simulink model "CabinGuard_MATLAB_simulation"  (R2024a)
settings: Solver=ode4  StartTime=0.0  StopTime=45  FixedStep=0.01  RelTol=1e-3
undefined symbols (not defined in the file or in its folder): ca_a_comf, ca_a_lo, ca_absvel, ca_clear, ca_d0, ca_det, ca_edge, ca_ego_id, ca_go_phase, ca_hw, ca_jdn, ca_jup, ca_kfeas, ca_lka_in, ca_lka_out, ca_lw0, ca_min_shift, ca_plant, ca_psi0, ca_pv, ca_sys, ca_t_act, ca_v0, ca_vlat, ca_wn, ca_X0, ca_Y0, driving, matlabshared
libraries: simulink x102, drivingscenarioandsensors x5, autolibshared x2, mpcadaslib x1, slpidlib x1
(part 4 of 4)

== system CabinGuard_MATLAB_simulation/GNC/Perception/C2_4 ==
  x : Inport
  y : Inport  Port=2
  vx : Inport  Port=3
  vy : Inport  Port=4
  v : Inport  Port=5
  kap : Inport  Port=6
  vm : Inport  Port=7
  xf : Inport  Port=8
  ASw : Switch  Criteria=u2 ~= 0  SaturateOnIntegerOverflow=off  InputSameDT=off
  AbsK : Constant  Value=ca_absvel
  AbsVm : Product  Inputs=**
  AbsY : Abs  SaturateOnIntegerOverflow=off
  Areq0 : Product  Inputs=*/
  B12 : Constant  Value=12
  Bsum : Sum
  D0 : Constant  Value=ca_d0
  Dx : Sum  Inputs=+-
  DxS : Saturate  UpperLimit=inf  LowerLimit=0.5
  G3 : Gain  Gain=3
  Half : Gain  Gain=0.5
  HalfA : Gain  Gain=0.5
  InPath : Logic  Inputs=3  AllPortsSameDT=off  OutDataTypeStr=boolean
  InW : simulink/Logic and Bit Operations/Compare To Constant  relop=<  const=ca_hw  OutDataTypeStr=boolean
  KX2 : Product  Inputs=**
  NegB : Gain  Gain=-1
  NegVx : Gain  Gain=-1
  Occ : Logic  Inputs=5  AllPortsSameDT=off  OutDataTypeStr=boolean
  Tm : Product  Inputs=*/
  Vc : Saturate  UpperLimit=inf  LowerLimit=0
  Vc2 : Product  Inputs=**
  VmS : Saturate  UpperLimit=inf  LowerLimit=1
  VxP : Saturate  UpperLimit=inf  LowerLimit=0
  VxRel : Sum  Inputs=+-
  VyT : Product  Inputs=**
  X2 : Product  Inputs=**
  XB : RelationalOperator  Operator=>  OutDataTypeStr=boolean  RndMeth=Simplest  InputSameDT=off
  XL : RelationalOperator  Operator=<  OutDataTypeStr=boolean  RndMeth=Simplest  InputSameDT=off
  XPos : simulink/Logic and Bit Operations/Compare To Constant  relop=>  const=0.5  OutDataTypeStr=boolean
  YP : Sum  Inputs=+-
  YPred : Sum
  YR1 : simulink/Logic and Bit Operations/Compare To Constant  relop=<  const=-0.9  OutDataTypeStr=boolean
  YR2 : simulink/Logic and Bit Operations/Compare To Constant  relop=>  const=-ca_clear+0.2  OutDataTypeStr=boolean
  Zero : Constant  Value=0
  areq : Outport
  occ : Outport  Port=2
  wires:
  AbsK/1 -> AbsVm/2
  xf/1 -> XL/2
  vm/1 -> VmS/1, AbsVm/1
  VxRel/1 -> NegVx/1, VxP/1
  vy/1 -> VyT/1
  vx/1 -> VxRel/1
  D0/1 -> Dx/2
  AbsVm/1 -> VxRel/2
  VmS/1 -> Tm/2
  ASw/1 -> areq/1
  y/1 -> YP/1
  x/1 -> Dx/1, XB/1, XPos/1, Tm/1, X2/2, XL/1, X2/1
  NegVx/1 -> Vc/1
  DxS/1 -> Areq0/2
  Dx/1 -> DxS/1
  Tm/1 -> VyT/2
  v/1 -> InPath/1, Occ/1
  kap/1 -> KX2/1
  X2/1 -> KX2/2
  VxP/1 -> G3/1
  YR2/1 -> Occ/3
  YR1/1 -> Occ/2
  XL/1 -> Occ/4
  Vc/1 -> Vc2/2, Vc2/1
  VyT/1 -> YPred/2
  NegB/1 -> XB/2
  KX2/1 -> Half/1
  G3/1 -> Bsum/1
  Areq0/1 -> HalfA/1
  B12/1 -> Bsum/2
  Vc2/1 -> Areq0/1
  Half/1 -> YP/2
  AbsY/1 -> InW/1
  Bsum/1 -> NegB/1
  YP/1 -> YPred/1, YR2/1, YR1/1
  YPred/1 -> AbsY/1
  XB/1 -> Occ/5
  Zero/1 -> ASw/3
  XPos/1 -> InPath/2
  Occ/1 -> occ/1
  HalfA/1 -> ASw/1
  InW/1 -> InPath/3
  InPath/1 -> ASw/2

== system CabinGuard_MATLAB_simulation/GNC/Perception/C2_5 ==
  x : Inport
  y : Inport  Port=2
  vx : Inport  Port=3
  vy : Inport  Port=4
  v : Inport  Port=5
  kap : Inport  Port=6
  vm : Inport  Port=7
  xf : Inport  Port=8
  ASw : Switch  Criteria=u2 ~= 0  SaturateOnIntegerOverflow=off  InputSameDT=off
  AbsK : Constant  Value=ca_absvel
  AbsVm : Product  Inputs=**
  AbsY : Abs  SaturateOnIntegerOverflow=off
  Areq0 : Product  Inputs=*/
  B12 : Constant  Value=12
  Bsum : Sum
  D0 : Constant  Value=ca_d0
  Dx : Sum  Inputs=+-
  DxS : Saturate  UpperLimit=inf  LowerLimit=0.5
  G3 : Gain  Gain=3
  Half : Gain  Gain=0.5
  HalfA : Gain  Gain=0.5
  InPath : Logic  Inputs=3  AllPortsSameDT=off  OutDataTypeStr=boolean
  InW : simulink/Logic and Bit Operations/Compare To Constant  relop=<  const=ca_hw  OutDataTypeStr=boolean
  KX2 : Product  Inputs=**
  NegB : Gain  Gain=-1
  NegVx : Gain  Gain=-1
  Occ : Logic  Inputs=5  AllPortsSameDT=off  OutDataTypeStr=boolean
  Tm : Product  Inputs=*/
  Vc : Saturate  UpperLimit=inf  LowerLimit=0
  Vc2 : Product  Inputs=**
  VmS : Saturate  UpperLimit=inf  LowerLimit=1
  VxP : Saturate  UpperLimit=inf  LowerLimit=0
  VxRel : Sum  Inputs=+-
  VyT : Product  Inputs=**
  X2 : Product  Inputs=**
  XB : RelationalOperator  Operator=>  OutDataTypeStr=boolean  RndMeth=Simplest  InputSameDT=off
  XL : RelationalOperator  Operator=<  OutDataTypeStr=boolean  RndMeth=Simplest  InputSameDT=off
  XPos : simulink/Logic and Bit Operations/Compare To Constant  relop=>  const=0.5  OutDataTypeStr=boolean
  YP : Sum  Inputs=+-
  YPred : Sum
  YR1 : simulink/Logic and Bit Operations/Compare To Constant  relop=<  const=-0.9  OutDataTypeStr=boolean
  YR2 : simulink/Logic and Bit Operations/Compare To Constant  relop=>  const=-ca_clear+0.2  OutDataTypeStr=boolean
  Zero : Constant  Value=0
  areq : Outport
  occ : Outport  Port=2
  wires:
  x/1 -> Dx/1, XB/1, XL/1, XPos/1, X2/2, Tm/1, X2/1
  VxRel/1 -> VxP/1, NegVx/1
  X2/1 -> KX2/2
  AbsK/1 -> AbsVm/2
  y/1 -> YP/1
  vx/1 -> VxRel/1
  kap/1 -> KX2/1
  vm/1 -> AbsVm/1, VmS/1
  AbsY/1 -> InW/1
  AbsVm/1 -> VxRel/2
  VmS/1 -> Tm/2
  Bsum/1 -> NegB/1
  D0/1 -> Dx/2
  xf/1 -> XL/2
  NegVx/1 -> Vc/1
  Dx/1 -> DxS/1
  vy/1 -> VyT/1
  Vc/1 -> Vc2/2, Vc2/1
  Tm/1 -> VyT/2
  VxP/1 -> G3/1
  XL/1 -> Occ/4
  VyT/1 -> YPred/2
  KX2/1 -> Half/1
  G3/1 -> Bsum/1
  B12/1 -> Bsum/2
  Vc2/1 -> Areq0/1
  DxS/1 -> Areq0/2
  InW/1 -> InPath/3
  HalfA/1 -> ASw/1
  Half/1 -> YP/2
  Areq0/1 -> HalfA/1
  YP/1 -> YPred/1, YR2/1, YR1/1
  NegB/1 -> XB/2
  v/1 -> InPath/1, Occ/1
  YR1/1 -> Occ/2
  YPred/1 -> AbsY/1
  YR2/1 -> Occ/3
  XB/1 -> Occ/5
  Occ/1 -> occ/1
  XPos/1 -> InPath/2
  InPath/1 -> ASw/2
  Zero/1 -> ASw/3
  ASw/1 -> areq/1

== system CabinGuard_MATLAB_simulation/GNC/Perception/C2_6 ==
  x : Inport
  y : Inport  Port=2
  vx : Inport  Port=3
  vy : Inport  Port=4
  v : Inport  Port=5
  kap : Inport  Port=6
  vm : Inport  Port=7
  xf : Inport  Port=8
  ASw : Switch  Criteria=u2 ~= 0  SaturateOnIntegerOverflow=off  InputSameDT=off
  AbsK : Constant  Value=ca_absvel
  AbsVm : Product  Inputs=**
  AbsY : Abs  SaturateOnIntegerOverflow=off
  Areq0 : Product  Inputs=*/
  B12 : Constant  Value=12
  Bsum : Sum
  D0 : Constant  Value=ca_d0
  Dx : Sum  Inputs=+-
  DxS : Saturate  UpperLimit=inf  LowerLimit=0.5
  G3 : Gain  Gain=3
  Half : Gain  Gain=0.5
  HalfA : Gain  Gain=0.5
  InPath : Logic  Inputs=3  AllPortsSameDT=off  OutDataTypeStr=boolean
  InW : simulink/Logic and Bit Operations/Compare To Constant  relop=<  const=ca_hw  OutDataTypeStr=boolean
  KX2 : Product  Inputs=**
  NegB : Gain  Gain=-1
  NegVx : Gain  Gain=-1
  Occ : Logic  Inputs=5  AllPortsSameDT=off  OutDataTypeStr=boolean
  Tm : Product  Inputs=*/
  Vc : Saturate  UpperLimit=inf  LowerLimit=0
  Vc2 : Product  Inputs=**
  VmS : Saturate  UpperLimit=inf  LowerLimit=1
  VxP : Saturate  UpperLimit=inf  LowerLimit=0
  VxRel : Sum  Inputs=+-
  VyT : Product  Inputs=**
  X2 : Product  Inputs=**
  XB : RelationalOperator  Operator=>  OutDataTypeStr=boolean  RndMeth=Simplest  InputSameDT=off
  XL : RelationalOperator  Operator=<  OutDataTypeStr=boolean  RndMeth=Simplest  InputSameDT=off
  XPos : simulink/Logic and Bit Operations/Compare To Constant  relop=>  const=0.5  OutDataTypeStr=boolean
  YP : Sum  Inputs=+-
  YPred : Sum
  YR1 : simulink/Logic and Bit Operations/Compare To Constant  relop=<  const=-0.9  OutDataTypeStr=boolean
  YR2 : simulink/Logic and Bit Operations/Compare To Constant  relop=>  const=-ca_clear+0.2  OutDataTypeStr=boolean
  Zero : Constant  Value=0
  areq : Outport
  occ : Outport  Port=2
  wires:
  AbsK/1 -> AbsVm/2
  kap/1 -> KX2/1
  vm/1 -> AbsVm/1, VmS/1
  x/1 -> Dx/1, XB/1, XL/1, Tm/1, XPos/1, X2/1, X2/2
  y/1 -> YP/1
  vx/1 -> VxRel/1
  DxS/1 -> Areq0/2
  AbsVm/1 -> VxRel/2
  VmS/1 -> Tm/2
  Vc/1 -> Vc2/2, Vc2/1
  D0/1 -> Dx/2
  VxRel/1 -> VxP/1, NegVx/1
  NegB/1 -> XB/2
  xf/1 -> XL/2
  InPath/1 -> ASw/2
  NegVx/1 -> Vc/1
  Dx/1 -> DxS/1
  v/1 -> InPath/1, Occ/1
  vy/1 -> VyT/1
  VyT/1 -> YPred/2
  Tm/1 -> VyT/2
  X2/1 -> KX2/2
  VxP/1 -> G3/1
  InW/1 -> InPath/3
  Occ/1 -> occ/1
  XL/1 -> Occ/4
  YP/1 -> YPred/1, YR2/1, YR1/1
  KX2/1 -> Half/1
  Half/1 -> YP/2
  G3/1 -> Bsum/1
  B12/1 -> Bsum/2
  ASw/1 -> areq/1
  Vc2/1 -> Areq0/1
  Bsum/1 -> NegB/1
  Areq0/1 -> HalfA/1
  YPred/1 -> AbsY/1
  YR1/1 -> Occ/2
  Zero/1 -> ASw/3
  YR2/1 -> Occ/3
  XB/1 -> Occ/5
  XPos/1 -> InPath/2
  AbsY/1 -> InW/1
  HalfA/1 -> ASw/1

== system CabinGuard_MATLAB_simulation/GNC/Perception/C3_1 ==
  x : Inport
  y : Inport  Port=2
  vx : Inport  Port=3
  vy : Inport  Port=4
  v : Inport  Port=5
  kap : Inport  Port=6
  vm : Inport  Port=7
  xf : Inport  Port=8
  ASw : Switch  Criteria=u2 ~= 0  SaturateOnIntegerOverflow=off  InputSameDT=off
  AbsK : Constant  Value=ca_absvel
  AbsVm : Product  Inputs=**
  AbsY : Abs  SaturateOnIntegerOverflow=off
  Areq0 : Product  Inputs=*/
  B12 : Constant  Value=12
  Bsum : Sum
  D0 : Constant  Value=ca_d0
  Dx : Sum  Inputs=+-
  DxS : Saturate  UpperLimit=inf  LowerLimit=0.5
  G3 : Gain  Gain=3
  Half : Gain  Gain=0.5
  HalfA : Gain  Gain=0.5
  InPath : Logic  Inputs=3  AllPortsSameDT=off  OutDataTypeStr=boolean
  InW : simulink/Logic and Bit Operations/Compare To Constant  relop=<  const=ca_hw  OutDataTypeStr=boolean
  KX2 : Product  Inputs=**
  NegB : Gain  Gain=-1
  NegVx : Gain  Gain=-1
  Occ : Logic  Inputs=5  AllPortsSameDT=off  OutDataTypeStr=boolean
  Tm : Product  Inputs=*/
  Vc : Saturate  UpperLimit=inf  LowerLimit=0
  Vc2 : Product  Inputs=**
  VmS : Saturate  UpperLimit=inf  LowerLimit=1
  VxP : Saturate  UpperLimit=inf  LowerLimit=0
  VxRel : Sum  Inputs=+-
  VyT : Product  Inputs=**
  X2 : Product  Inputs=**
  XB : RelationalOperator  Operator=>  OutDataTypeStr=boolean  RndMeth=Simplest  InputSameDT=off
  XL : RelationalOperator  Operator=<  OutDataTypeStr=boolean  RndMeth=Simplest  InputSameDT=off
  XPos : simulink/Logic and Bit Operations/Compare To Constant  relop=>  const=0.5  OutDataTypeStr=boolean
  YP : Sum  Inputs=+-
  YPred : Sum
  YR1 : simulink/Logic and Bit Operations/Compare To Constant  relop=<  const=-0.9  OutDataTypeStr=boolean
  YR2 : simulink/Logic and Bit Operations/Compare To Constant  relop=>  const=-ca_clear+0.2  OutDataTypeStr=boolean
  Zero : Constant  Value=0
  areq : Outport
  occ : Outport  Port=2
  wires:
  VxRel/1 -> VxP/1, NegVx/1
  x/1 -> Dx/1, XPos/1, Tm/1, XB/1, X2/2, X2/1, XL/1
  InW/1 -> InPath/3
  AbsK/1 -> AbsVm/2
  y/1 -> YP/1
  Vc2/1 -> Areq0/1
  vx/1 -> VxRel/1
  KX2/1 -> Half/1
  vm/1 -> VmS/1, AbsVm/1
  AbsY/1 -> InW/1
  AbsVm/1 -> VxRel/2
  VmS/1 -> Tm/2
  Bsum/1 -> NegB/1
  D0/1 -> Dx/2
  NegB/1 -> XB/2
  xf/1 -> XL/2
  NegVx/1 -> Vc/1
  XB/1 -> Occ/5
  Dx/1 -> DxS/1
  Occ/1 -> occ/1
  vy/1 -> VyT/1
  Vc/1 -> Vc2/2, Vc2/1
  Tm/1 -> VyT/2
  YR1/1 -> Occ/2
  YPred/1 -> AbsY/1
  kap/1 -> KX2/1
  YR2/1 -> Occ/3
  X2/1 -> KX2/2
  Zero/1 -> ASw/3
  VxP/1 -> G3/1
  XL/1 -> Occ/4
  ASw/1 -> areq/1
  InPath/1 -> ASw/2
  VyT/1 -> YPred/2
  G3/1 -> Bsum/1
  B12/1 -> Bsum/2
  DxS/1 -> Areq0/2
  Half/1 -> YP/2
  Areq0/1 -> HalfA/1
  YP/1 -> YPred/1, YR2/1, YR1/1
  v/1 -> InPath/1, Occ/1
  XPos/1 -> InPath/2
  HalfA/1 -> ASw/1

== system CabinGuard_MATLAB_simulation/GNC/Perception/C3_2 ==
  x : Inport
  y : Inport  Port=2
  vx : Inport  Port=3
  vy : Inport  Port=4
  v : Inport  Port=5
  kap : Inport  Port=6
  vm : Inport  Port=7
  xf : Inport  Port=8
  ASw : Switch  Criteria=u2 ~= 0  SaturateOnIntegerOverflow=off  InputSameDT=off
  AbsK : Constant  Value=ca_absvel
  AbsVm : Product  Inputs=**
  AbsY : Abs  SaturateOnIntegerOverflow=off
  Areq0 : Product  Inputs=*/
  B12 : Constant  Value=12
  Bsum : Sum
  D0 : Constant  Value=ca_d0
  Dx : Sum  Inputs=+-
  DxS : Saturate  UpperLimit=inf  LowerLimit=0.5
  G3 : Gain  Gain=3
  Half : Gain  Gain=0.5
  HalfA : Gain  Gain=0.5
  InPath : Logic  Inputs=3  AllPortsSameDT=off  OutDataTypeStr=boolean
  InW : simulink/Logic and Bit Operations/Compare To Constant  relop=<  const=ca_hw  OutDataTypeStr=boolean
  KX2 : Product  Inputs=**
  NegB : Gain  Gain=-1
  NegVx : Gain  Gain=-1
  Occ : Logic  Inputs=5  AllPortsSameDT=off  OutDataTypeStr=boolean
  Tm : Product  Inputs=*/
  Vc : Saturate  UpperLimit=inf  LowerLimit=0
  Vc2 : Product  Inputs=**
  VmS : Saturate  UpperLimit=inf  LowerLimit=1
  VxP : Saturate  UpperLimit=inf  LowerLimit=0
  VxRel : Sum  Inputs=+-
  VyT : Product  Inputs=**
  X2 : Product  Inputs=**
  XB : RelationalOperator  Operator=>  OutDataTypeStr=boolean  RndMeth=Simplest  InputSameDT=off
  XL : RelationalOperator  Operator=<  OutDataTypeStr=boolean  RndMeth=Simplest  InputSameDT=off
  XPos : simulink/Logic and Bit Operations/Compare To Constant  relop=>  const=0.5  OutDataTypeStr=boolean
  YP : Sum  Inputs=+-
  YPred : Sum
  YR1 : simulink/Logic and Bit Operations/Compare To Constant  relop=<  const=-0.9  OutDataTypeStr=boolean
  YR2 : simulink/Logic and Bit Operations/Compare To Constant  relop=>  const=-ca_clear+0.2  OutDataTypeStr=boolean
  Zero : Constant  Value=0
  areq : Outport
  occ : Outport  Port=2
  wires:
  y/1 -> YP/1
  Tm/1 -> VyT/2
  vx/1 -> VxRel/1
  AbsK/1 -> AbsVm/2
  vm/1 -> AbsVm/1, VmS/1
  HalfA/1 -> ASw/1
  x/1 -> Dx/1, XPos/1, XL/1, X2/2, X2/1, Tm/1, XB/1
  AbsVm/1 -> VxRel/2
  VmS/1 -> Tm/2
  VxP/1 -> G3/1
  X2/1 -> KX2/2
  VxRel/1 -> NegVx/1, VxP/1
  Bsum/1 -> NegB/1
  D0/1 -> Dx/2
  xf/1 -> XL/2
  Occ/1 -> occ/1
  B12/1 -> Bsum/2
  NegVx/1 -> Vc/1
  YP/1 -> YPred/1, YR1/1, YR2/1
  Dx/1 -> DxS/1
  vy/1 -> VyT/1
  kap/1 -> KX2/1
  XB/1 -> Occ/5
  Half/1 -> YP/2
  G3/1 -> Bsum/1
  XL/1 -> Occ/4
  Vc2/1 -> Areq0/1
  Vc/1 -> Vc2/2, Vc2/1
  YR2/1 -> Occ/3
  VyT/1 -> YPred/2
  KX2/1 -> Half/1
  DxS/1 -> Areq0/2
  Areq0/1 -> HalfA/1
  NegB/1 -> XB/2
  v/1 -> InPath/1, Occ/1
  YPred/1 -> AbsY/1
  AbsY/1 -> InW/1
  YR1/1 -> Occ/2
  XPos/1 -> InPath/2
  InW/1 -> InPath/3
  InPath/1 -> ASw/2
  ASw/1 -> areq/1
  Zero/1 -> ASw/3

== system CabinGuard_MATLAB_simulation/GNC/Perception/C3_3 ==
  x : Inport
  y : Inport  Port=2
  vx : Inport  Port=3
  vy : Inport  Port=4
  v : Inport  Port=5
  kap : Inport  Port=6
  vm : Inport  Port=7
  xf : Inport  Port=8
  ASw : Switch  Criteria=u2 ~= 0  SaturateOnIntegerOverflow=off  InputSameDT=off
  AbsK : Constant  Value=ca_absvel
  AbsVm : Product  Inputs=**
  AbsY : Abs  SaturateOnIntegerOverflow=off
  Areq0 : Product  Inputs=*/
  B12 : Constant  Value=12
  Bsum : Sum
  D0 : Constant  Value=ca_d0
  Dx : Sum  Inputs=+-
  DxS : Saturate  UpperLimit=inf  LowerLimit=0.5
  G3 : Gain  Gain=3
  Half : Gain  Gain=0.5
  HalfA : Gain  Gain=0.5
  InPath : Logic  Inputs=3  AllPortsSameDT=off  OutDataTypeStr=boolean
  InW : simulink/Logic and Bit Operations/Compare To Constant  relop=<  const=ca_hw  OutDataTypeStr=boolean
  KX2 : Product  Inputs=**
  NegB : Gain  Gain=-1
  NegVx : Gain  Gain=-1
  Occ : Logic  Inputs=5  AllPortsSameDT=off  OutDataTypeStr=boolean
  Tm : Product  Inputs=*/
  Vc : Saturate  UpperLimit=inf  LowerLimit=0
  Vc2 : Product  Inputs=**
  VmS : Saturate  UpperLimit=inf  LowerLimit=1
  VxP : Saturate  UpperLimit=inf  LowerLimit=0
  VxRel : Sum  Inputs=+-
  VyT : Product  Inputs=**
  X2 : Product  Inputs=**
  XB : RelationalOperator  Operator=>  OutDataTypeStr=boolean  RndMeth=Simplest  InputSameDT=off
  XL : RelationalOperator  Operator=<  OutDataTypeStr=boolean  RndMeth=Simplest  InputSameDT=off
  XPos : simulink/Logic and Bit Operations/Compare To Constant  relop=>  const=0.5  OutDataTypeStr=boolean
  YP : Sum  Inputs=+-
  YPred : Sum
  YR1 : simulink/Logic and Bit Operations/Compare To Constant  relop=<  const=-0.9  OutDataTypeStr=boolean
  YR2 : simulink/Logic and Bit Operations/Compare To Constant  relop=>  const=-ca_clear+0.2  OutDataTypeStr=boolean
  Zero : Constant  Value=0
  areq : Outport
  occ : Outport  Port=2
  wires:
  v/1 -> InPath/1, Occ/1
  vm/1 -> AbsVm/1, VmS/1
  AbsK/1 -> AbsVm/2
  vx/1 -> VxRel/1
  x/1 -> Dx/1, XPos/1, XL/1, Tm/1, XB/1, X2/2, X2/1
  AbsVm/1 -> VxRel/2
  VmS/1 -> Tm/2
  Dx/1 -> DxS/1
  D0/1 -> Dx/2
  XB/1 -> Occ/5
  VyT/1 -> YPred/2
  X2/1 -> KX2/2
  VxRel/1 -> VxP/1, NegVx/1
  kap/1 -> KX2/1
  xf/1 -> XL/2
  Occ/1 -> occ/1
  YR1/1 -> Occ/2
  NegVx/1 -> Vc/1
  y/1 -> YP/1
  vy/1 -> VyT/1
  Tm/1 -> VyT/2
  VxP/1 -> G3/1
  XL/1 -> Occ/4
  Vc2/1 -> Areq0/1
  Vc/1 -> Vc2/2, Vc2/1
  InPath/1 -> ASw/2
  InW/1 -> InPath/3
  HalfA/1 -> ASw/1
  KX2/1 -> Half/1
  G3/1 -> Bsum/1
  B12/1 -> Bsum/2
  DxS/1 -> Areq0/2
  Half/1 -> YP/2
  Bsum/1 -> NegB/1
  AbsY/1 -> InW/1
  Areq0/1 -> HalfA/1
  XPos/1 -> InPath/2
  YPred/1 -> AbsY/1
  NegB/1 -> XB/2
  YP/1 -> YR2/1, YR1/1, YPred/1
  YR2/1 -> Occ/3
  Zero/1 -> ASw/3
  ASw/1 -> areq/1

== system CabinGuard_MATLAB_simulation/GNC/Perception/C3_4 ==
  x : Inport
  y : Inport  Port=2
  vx : Inport  Port=3
  vy : Inport  Port=4
  v : Inport  Port=5
  kap : Inport  Port=6
  vm : Inport  Port=7
  xf : Inport  Port=8
  ASw : Switch  Criteria=u2 ~= 0  SaturateOnIntegerOverflow=off  InputSameDT=off
  AbsK : Constant  Value=ca_absvel
  AbsVm : Product  Inputs=**
  AbsY : Abs  SaturateOnIntegerOverflow=off
  Areq0 : Product  Inputs=*/
  B12 : Constant  Value=12
  Bsum : Sum
  D0 : Constant  Value=ca_d0
  Dx : Sum  Inputs=+-
  DxS : Saturate  UpperLimit=inf  LowerLimit=0.5
  G3 : Gain  Gain=3
  Half : Gain  Gain=0.5
  HalfA : Gain  Gain=0.5
  InPath : Logic  Inputs=3  AllPortsSameDT=off  OutDataTypeStr=boolean
  InW : simulink/Logic and Bit Operations/Compare To Constant  relop=<  const=ca_hw  OutDataTypeStr=boolean
  KX2 : Product  Inputs=**
  NegB : Gain  Gain=-1
  NegVx : Gain  Gain=-1
  Occ : Logic  Inputs=5  AllPortsSameDT=off  OutDataTypeStr=boolean
  Tm : Product  Inputs=*/
  Vc : Saturate  UpperLimit=inf  LowerLimit=0
  Vc2 : Product  Inputs=**
  VmS : Saturate  UpperLimit=inf  LowerLimit=1
  VxP : Saturate  UpperLimit=inf  LowerLimit=0
  VxRel : Sum  Inputs=+-
  VyT : Product  Inputs=**
  X2 : Product  Inputs=**
  XB : RelationalOperator  Operator=>  OutDataTypeStr=boolean  RndMeth=Simplest  InputSameDT=off
  XL : RelationalOperator  Operator=<  OutDataTypeStr=boolean  RndMeth=Simplest  InputSameDT=off
  XPos : simulink/Logic and Bit Operations/Compare To Constant  relop=>  const=0.5  OutDataTypeStr=boolean
  YP : Sum  Inputs=+-
  YPred : Sum
  YR1 : simulink/Logic and Bit Operations/Compare To Constant  relop=<  const=-0.9  OutDataTypeStr=boolean
  YR2 : simulink/Logic and Bit Operations/Compare To Constant  relop=>  const=-ca_clear+0.2  OutDataTypeStr=boolean
  Zero : Constant  Value=0
  areq : Outport
  occ : Outport  Port=2
  wires:
  AbsK/1 -> AbsVm/2
  AbsVm/1 -> VxRel/2
  v/1 -> InPath/1, Occ/1
  vm/1 -> AbsVm/1, VmS/1
  vx/1 -> VxRel/1
  x/1 -> XB/1, XPos/1, XL/1, Tm/1, X2/1, X2/2, Dx/1
  VyT/1 -> YPred/2
  VxP/1 -> G3/1
  X2/1 -> KX2/2
  VxRel/1 -> NegVx/1, VxP/1
  VmS/1 -> Tm/2
  Areq0/1 -> HalfA/1
  Dx/1 -> DxS/1
  D0/1 -> Dx/2
  y/1 -> YP/1
  kap/1 -> KX2/1
  vy/1 -> VyT/1
  xf/1 -> XL/2
  Occ/1 -> occ/1
  NegVx/1 -> Vc/1
  Tm/1 -> VyT/2
  XL/1 -> Occ/4
  DxS/1 -> Areq0/2
  Vc2/1 -> Areq0/1
  Vc/1 -> Vc2/2, Vc2/1
  InW/1 -> InPath/3
  KX2/1 -> Half/1
  G3/1 -> Bsum/1
  Bsum/1 -> NegB/1
  B12/1 -> Bsum/2
  Half/1 -> YP/2
  XPos/1 -> InPath/2
  YP/1 -> YPred/1, YR2/1, YR1/1
  NegB/1 -> XB/2
  YPred/1 -> AbsY/1
  YR1/1 -> Occ/2
  YR2/1 -> Occ/3
  XB/1 -> Occ/5
  AbsY/1 -> InW/1
  InPath/1 -> ASw/2
  HalfA/1 -> ASw/1
  Zero/1 -> ASw/3
  ASw/1 -> areq/1

== system CabinGuard_MATLAB_simulation/GNC/Perception/C3_5 ==
  x : Inport
  y : Inport  Port=2
  vx : Inport  Port=3
  vy : Inport  Port=4
  v : Inport  Port=5
  kap : Inport  Port=6
  vm : Inport  Port=7
  xf : Inport  Port=8
  ASw : Switch  Criteria=u2 ~= 0  SaturateOnIntegerOverflow=off  InputSameDT=off
  AbsK : Constant  Value=ca_absvel
  AbsVm : Product  Inputs=**
  AbsY : Abs  SaturateOnIntegerOverflow=off
  Areq0 : Product  Inputs=*/
  B12 : Constant  Value=12
  Bsum : Sum
  D0 : Constant  Value=ca_d0
  Dx : Sum  Inputs=+-
  DxS : Saturate  UpperLimit=inf  LowerLimit=0.5
  G3 : Gain  Gain=3
  Half : Gain  Gain=0.5
  HalfA : Gain  Gain=0.5
  InPath : Logic  Inputs=3  AllPortsSameDT=off  OutDataTypeStr=boolean
  InW : simulink/Logic and Bit Operations/Compare To Constant  relop=<  const=ca_hw  OutDataTypeStr=boolean
  KX2 : Product  Inputs=**
  NegB : Gain  Gain=-1
  NegVx : Gain  Gain=-1
  Occ : Logic  Inputs=5  AllPortsSameDT=off  OutDataTypeStr=boolean
  Tm : Product  Inputs=*/
  Vc : Saturate  UpperLimit=inf  LowerLimit=0
  Vc2 : Product  Inputs=**
  VmS : Saturate  UpperLimit=inf  LowerLimit=1
  VxP : Saturate  UpperLimit=inf  LowerLimit=0
  VxRel : Sum  Inputs=+-
  VyT : Product  Inputs=**
  X2 : Product  Inputs=**
  XB : RelationalOperator  Operator=>  OutDataTypeStr=boolean  RndMeth=Simplest  InputSameDT=off
  XL : RelationalOperator  Operator=<  OutDataTypeStr=boolean  RndMeth=Simplest  InputSameDT=off
  XPos : simulink/Logic and Bit Operations/Compare To Constant  relop=>  const=0.5  OutDataTypeStr=boolean
  YP : Sum  Inputs=+-
  YPred : Sum
  YR1 : simulink/Logic and Bit Operations/Compare To Constant  relop=<  const=-0.9  OutDataTypeStr=boolean
  YR2 : simulink/Logic and Bit Operations/Compare To Constant  relop=>  const=-ca_clear+0.2  OutDataTypeStr=boolean
  Zero : Constant  Value=0
  areq : Outport
  occ : Outport  Port=2
  wires:
  AbsVm/1 -> VxRel/2
  Half/1 -> YP/2
  AbsK/1 -> AbsVm/2
  Areq0/1 -> HalfA/1
  x/1 -> XB/1, XPos/1, Dx/1, Tm/1, X2/2, XL/1, X2/1
  v/1 -> InPath/1, Occ/1
  D0/1 -> Dx/2
  vx/1 -> VxRel/1
  AbsY/1 -> InW/1
  Dx/1 -> DxS/1
  vm/1 -> AbsVm/1, VmS/1
  VmS/1 -> Tm/2
  XL/1 -> Occ/4
  VxRel/1 -> VxP/1, NegVx/1
  xf/1 -> XL/2
  VyT/1 -> YPred/2
  NegVx/1 -> Vc/1
  Bsum/1 -> NegB/1
  vy/1 -> VyT/1
  Tm/1 -> VyT/2
  kap/1 -> KX2/1
  Occ/1 -> occ/1
  X2/1 -> KX2/2
  XB/1 -> Occ/5
  VxP/1 -> G3/1
  HalfA/1 -> ASw/1
  Vc/1 -> Vc2/2, Vc2/1
  KX2/1 -> Half/1
  y/1 -> YP/1
  B12/1 -> Bsum/2
  G3/1 -> Bsum/1
  InPath/1 -> ASw/2
  Vc2/1 -> Areq0/1
  DxS/1 -> Areq0/2
  YP/1 -> YPred/1, YR2/1, YR1/1
  NegB/1 -> XB/2
  YPred/1 -> AbsY/1
  YR1/1 -> Occ/2
  YR2/1 -> Occ/3
  Zero/1 -> ASw/3
  XPos/1 -> InPath/2
  InW/1 -> InPath/3
  ASw/1 -> areq/1

== system CabinGuard_MATLAB_simulation/GNC/Perception/C3_6 ==
  x : Inport
  y : Inport  Port=2
  vx : Inport  Port=3
  vy : Inport  Port=4
  v : Inport  Port=5
  kap : Inport  Port=6
  vm : Inport  Port=7
  xf : Inport  Port=8
  ASw : Switch  Criteria=u2 ~= 0  SaturateOnIntegerOverflow=off  InputSameDT=off
  AbsK : Constant  Value=ca_absvel
  AbsVm : Product  Inputs=**
  AbsY : Abs  SaturateOnIntegerOverflow=off
  Areq0 : Product  Inputs=*/
  B12 : Constant  Value=12
  Bsum : Sum
  D0 : Constant  Value=ca_d0
  Dx : Sum  Inputs=+-
  DxS : Saturate  UpperLimit=inf  LowerLimit=0.5
  G3 : Gain  Gain=3
  Half : Gain  Gain=0.5
  HalfA : Gain  Gain=0.5
  InPath : Logic  Inputs=3  AllPortsSameDT=off  OutDataTypeStr=boolean
  InW : simulink/Logic and Bit Operations/Compare To Constant  relop=<  const=ca_hw  OutDataTypeStr=boolean
  KX2 : Product  Inputs=**
  NegB : Gain  Gain=-1
  NegVx : Gain  Gain=-1
  Occ : Logic  Inputs=5  AllPortsSameDT=off  OutDataTypeStr=boolean
  Tm : Product  Inputs=*/
  Vc : Saturate  UpperLimit=inf  LowerLimit=0
  Vc2 : Product  Inputs=**
  VmS : Saturate  UpperLimit=inf  LowerLimit=1
  VxP : Saturate  UpperLimit=inf  LowerLimit=0
  VxRel : Sum  Inputs=+-
  VyT : Product  Inputs=**
  X2 : Product  Inputs=**
  XB : RelationalOperator  Operator=>  OutDataTypeStr=boolean  RndMeth=Simplest  InputSameDT=off
  XL : RelationalOperator  Operator=<  OutDataTypeStr=boolean  RndMeth=Simplest  InputSameDT=off
  XPos : simulink/Logic and Bit Operations/Compare To Constant  relop=>  const=0.5  OutDataTypeStr=boolean
  YP : Sum  Inputs=+-
  YPred : Sum
  YR1 : simulink/Logic and Bit Operations/Compare To Constant  relop=<  const=-0.9  OutDataTypeStr=boolean
  YR2 : simulink/Logic and Bit Operations/Compare To Constant  relop=>  const=-ca_clear+0.2  OutDataTypeStr=boolean
  Zero : Constant  Value=0
  areq : Outport
  occ : Outport  Port=2
  wires:
  AbsVm/1 -> VxRel/2
  AbsK/1 -> AbsVm/2
  Areq0/1 -> HalfA/1
  x/1 -> XB/1, XL/1, XPos/1, Dx/1, Tm/1, X2/1, X2/2
  vx/1 -> VxRel/1
  AbsY/1 -> InW/1
  vm/1 -> AbsVm/1, VmS/1
  DxS/1 -> Areq0/2
  VmS/1 -> Tm/2
  HalfA/1 -> ASw/1
  Vc/1 -> Vc2/2, Vc2/1
  D0/1 -> Dx/2
  XL/1 -> Occ/4
  VxRel/1 -> NegVx/1, VxP/1
  xf/1 -> XL/2
  NegVx/1 -> Vc/1
  InPath/1 -> ASw/2
  Vc2/1 -> Areq0/1
  Dx/1 -> DxS/1
  vy/1 -> VyT/1
  Half/1 -> YP/2
  Tm/1 -> VyT/2
  kap/1 -> KX2/1
  X2/1 -> KX2/2
  XB/1 -> Occ/5
  VxP/1 -> G3/1
  VyT/1 -> YPred/2
  KX2/1 -> Half/1
  B12/1 -> Bsum/2
  G3/1 -> Bsum/1
  y/1 -> YP/1
  Bsum/1 -> NegB/1
  YP/1 -> YR2/1, YR1/1, YPred/1
  NegB/1 -> XB/2
  v/1 -> InPath/1, Occ/1
  YPred/1 -> AbsY/1
  YR1/1 -> Occ/2
  YR2/1 -> Occ/3
  Zero/1 -> ASw/3
  XPos/1 -> InPath/2
  Occ/1 -> occ/1
  InW/1 -> InPath/3
  ASw/1 -> areq/1

== matlab function CabinGuard_MATLAB_simulation/CabinGuard/Tel ==
  settings: updateMethod=DISCRETE  sampleTime=0.01
  data: t input; delivered output; ecall input; cls input; Pmax input; cell_up input; sms_up input
function delivered  = fcn(t, ecall, cls, Pmax, cell_up, sms_up)
% EMERGENCY MESSAGE TRANSPORT (MEC): cellular retries at +0, +1, +3, +7 s (backoff 1,2,4),
% then SMS, then retry every 30 s. The manoeuvre never waits for it.
% cls and Pmax are the (anonymized) message content; the signature/encryption are
% unit-tested in Python, here only delivery timing is simulated.
persistent trig t0 done idx tn
if isempty(trig)
    trig = false;  t0 = 0;  done = false;  idx = 1;  tn = 0;
end
if ecall > 0.5 && ~trig
    trig = true;  t0 = t;  tn = t;  idx = 1;
end
if trig && ~done && t >= tn
    if idx <= 4
        ok = cell_up > 0.5;
    elseif idx == 5
        ok = sms_up > 0.5;
    else
        ok = (cell_up > 0.5) || (sms_up > 0.5);
    end
    if ok
        done = true;
    else
        idx = idx + 1;
        offs = [0 1 3 7 8];
        if idx <= 5
            tn = t0 + offs(idx);
        else
            tn = t + 30;
        end
    end
end
delivered = double(done);
end

== matlab function CabinGuard_MATLAB_simulation/CabinGuard/Flt ==
  settings: updateMethod=DISCRETE  sampleTime=0.01
  data: t input; lam_f output; lam input; pv input; avail output; att output; cell_up output; sms_up output
function [lam_f, avail, att, cell_up, sms_up] = fcn(t, lam, pv)
% FAULT / ATTACK INJECTOR
%   fault id (pv(8)), starting at t_fault (pv(9)):
%    0 none            1 camera lost      2 IMU lost         3 seat sensor lost
%    4 host hang (handled in Host + Gateway)
%    5 forged command (bad MAC)           6 replayed command (stale freshness)
%    7 valid MAC but implausible decel    8 cellular down 60 s
%    9 camera blinded/spoofed (no pulse + closed eyes)
%   10 all bearers down 60 s             11 valid MAC but phase skipped
%   att = attacker frame [present; phase; decel; mac_ok; fresh_ok] at 10 Hz
lam_f = lam(:);
avail = [1; 1; 1];
att = zeros(5, 1);
cell_up = 1;  sms_up = 1;
fid = pv(8);  tf = pv(9);
on = (t >= tf);
tick = abs(t/0.1 - round(t/0.1)) < 1e-6;
switch fid
    case 1
        if on, avail(1) = 0; end
    case 2
        if on, avail(2) = 0; end
    case 3
        if on, avail(3) = 0; end
    case 5
        if on && tick, att = [1; 3; -4; 0; 1]; end
    case 6
        if on && tick, att = [1; 3; -3; 1; 0]; end
    case 7
        if on && tick, att = [1; 0; -6; 1; 1]; end
    case 8
        if on && t < tf + 60, cell_up = 0; end
    case 9
        if on, lam_f(1) = 6; lam_f(3) = 6; end
    case 10
        if on && t < tf + 60, cell_up = 0; sms_up = 0; end
    case 11
        if on && tick, att = [1; 3; -3; 1; 1]; end
end
end

== matlab function CabinGuard_MATLAB_simulation/CabinGuard/Det ==
  settings: updateMethod=DISCRETE  sampleTime=0.01
  data: t input; lam output; pv input; dp input
function lam = fcn(t, pv, dp)
% SURROGATE OF THE AI DETECTORS (replace with the real network output when it is connected).
%   Gives the log-evidence the Host expects: 4 branches (cardiac, vision, IMU/motion, seat/grip) x 2 classes (syncope, seizure).
%   lam = [S1 Z1 S2 Z2 S3 Z3 S4 Z4]'
%   pv(1) = incapacitation onset, pv(2) = event (0 none, 1 syncope, 2 seizure)
%   dp(1) = detector delay [s] after the onset, dp(2) = ramp time [s]
%   dp(3:5) = false alarm: start [s], duration [s], mode (0 none, 1 camera branches only, 2 all branches)
lam = zeros(8, 1);
ev = pv(2);  ton = pv(1);
dly = dp(1);  ramp = max(dp(2), 0.1);
if ev ~= 0 && t >= ton + dly
    g = min(1, (t - ton - dly) / ramp);
    k = min(max(round(ev), 1), 2);
    for b = 1:4
        lam(2*b - 2 + k) = 4 * g;
        lam(2*b - 2 + 3 - k) = -2 * g;
    end
end
if dp(5) > 0.5 && t >= dp(3) && t < dp(3) + dp(4)
    nb = 2;
    if dp(5) > 1.5, nb = 4; end
    for b = 1:nb
        lam(2*b - 1) = 4;  lam(2*b) = -2;
    end
end
end

== matlab function CabinGuard_MATLAB_simulation/CabinGuard/Drv ==
  settings: updateMethod=DISCRETE  sampleTime=0.01
  data: t input; steer output; y input; psi input; v input; pv input; a_drv output; tau output; brake_pedal output; clonic output; grip output
function [steer, a_drv, tau, brake_pedal, clonic, grip] = fcn(t, y, psi, v, pv)
% DRIVER + INCAPACITATION INJECTOR (kinematic-bicycle driver model)
%   outputs: steer (rad, front wheel), a_drv (m/s2 traction demand), tau (Nm, wheel torque),
%            brake_pedal (0/1), clonic (0/1, from motion features), grip (0 active, 1 off, 2 clenched)
L = 2.7;  wn = 0.8;  zt = 0.9;
t_on = pv(1);  ev = pv(2);  v0 = pv(3);  t_can = pv(10);  tonic = pv(14);
vs = max(v, 5);
drag = 0.5*1.2*0.7*v^2/1500 + 0.012*9.81;
% conscious driver: lane keeping + speed hold
steer = -(wn^2*L/vs^2)*y - (2*zt*wn*L/vs)*psi;
a_drv = min(2, max(-3, drag + 0.5*(v0 - v)));
tau = 1.5 + 20*abs(steer);
brake_pedal = 0;  clonic = 0;  grip = 0;

% conscious driver answering a false alarm
if ev == 0 && t_can > 0 && t >= t_can
    brake_pedal = 1;  tau = 6;  a_drv = -1.5;
end

if ev ~= 0 && t >= t_on
    te = t - t_on;
    if ev == 1                      % syncope: flaccid, hands off, pedal released
        steer = 0;  a_drv = 0;  tau = 0;  grip = 1;
    else                            % seizure
        if te < tonic               % tonic: clenched grip, wheel pushed, pedal held
            steer = 0.01;  a_drv = drag;  tau = 8;  grip = 2;
        else                        % clonic: 4 Hz jerking on wheel and pedal
            ph = 2*pi*4*(te - tonic);
            steer = 0.01 + 0.015*sin(ph);
            a_drv = drag + 1.0*sin(ph);
            tau = 8*sin(ph);
            clonic = 1;  grip = 2;
        end
    end
end
steer = max(-0.1, min(0.1, steer));
end

== matlab function CabinGuard_MATLAB_simulation/CabinGuard/Host ==
  settings: updateMethod=DISCRETE  sampleTime=0.01
  data: t input; hf output; lam input; avail input; tau input; grip input; clonic input; brake_pedal input; v input; pv input; F output; alert output; dmode output; Pmax output; cls output; ecall output; warn output; state output
function [hf, F, alert, dmode, Pmax, cls, ecall, warn, state] = fcn(t, lam, avail, tau, grip, clonic, brake_pedal, v, pv)
% EDGE HOST: bounded-evidence fusion (Eqs. 3-6), 2 s verification, two-sensor rule,
% camera interlock, degraded modes and the MRM state machine. Detector runs at 10 Hz.
%   state: 0 NORMAL, 1 ALERT, 2 HAZARD, 3 BRAKE, 4 STANDSTILL
%   dmode: 0 nominal, 1 camera lost, 2 IMU lost, 3 <2 sensors (no MRM), 4 seat lost
%   hf   : command frame [send; phase; decel_req; mac_ok; fresh_ok] (crypto outcome is
%          abstracted: the SecOC MAC/freshness are unit-tested in the Python code)
c = 3;  GAM = 0.85;  NW = 20;  TVER = 2;
lp = log([0.8 0.1 0.1]);                     % operational prior N, S, Z

persistent n buf vcnt st t_a cool dist_until Pm cl md wr last_ie
if isempty(n)
    n = 0;  buf = zeros(NW, 8);  vcnt = 0;  st = 0;  t_a = 0;
    cool = -1;  dist_until = -1;  Pm = 0;  cl = 0;  md = 0;  wr = 0;  last_ie = 0;
end
lam = lam(:);  avail = avail(:);
n = n + 1;
tick = (mod(n, 10) == 0);

if tick
    % cross-sensor interlock: camera claims an event while the wheel shows an upright,
    % steering driver -> distrust the camera for 10 s
    if max(lam(1:4)) >= 1 && tau > 1 && grip < 0.5 && clonic < 0.5
        dist_until = t + 10;
    end
    cam_ok = (avail(1) > 0.5) && (t >= dist_until);
    imu_ok = avail(2) > 0.5;
    seat_ok = avail(3) > 0.5;

    % Eq. (4): bounded evidence per branch (shifts both event classes together)
    lb = zeros(8, 1);
    for b = 1:4
        l2 = lam(2*b-1:2*b);
        m = max(0, max(l2) - c);
        lb(2*b-1:2*b) = max(-c, l2 - m);
    end
    bav = [cam_ok; cam_ok; imu_ok; seat_ok];  % cardiac+vision need camera
    for b = 1:4
        if ~bav(b), lb(2*b-1:2*b) = 0; end
    end
    buf = [buf(2:end, :); lb'];
    lbar = mean(buf, 1)';                     % average over last W = 2 s

    % Eq. (5): fused posterior
    sS = lbar(1) + lbar(3) + lbar(5) + lbar(7);
    sZ = lbar(2) + lbar(4) + lbar(6) + lbar(8);
    lg = [lp(1), lp(2) + sS, lp(3) + sZ];
    lg = lg - max(lg);
    p = exp(lg) / sum(exp(lg));
    [pe, ie] = max(p(2:3));

    % two physical sensors must agree (camera counts once)
    cols = [1 3 5 7] + (ie - 1);
    camAg = (lbar(cols(1)) >= 1) || (lbar(cols(2)) >= 1);
    nag = double(camAg) + double(lbar(cols(3)) >= 1) + double(lbar(cols(4)) >= 1);

    nav = double(cam_ok) + double(imu_ok) + double(seat_ok);
    if nav < 2
        md = 3;
    elseif avail(1) <= 0.5
        md = 1;
    elseif avail(2) <= 0.5
        md = 2;
    elseif avail(3) <= 0.5
        md = 4;
    else
        md = 0;
    end

    if ie ~= last_ie, vcnt = 0; end
    last_ie = ie;
    if pe >= GAM && nag >= 2 && t >= cool
        vcnt = vcnt + 1;
    else
        vcnt = 0;
    end
    cand = (vcnt >= TVER/0.1) && (nav >= 2) && (pv(15) > 0.5);
    wr = double((nav < 2) && (pe >= GAM));    % warn only, MRM forbidden
    Pm = pe;  cl = ie;

    % MRM state machine (design values of the paper)
    switch st
        case 0
            if cand, st = 1; t_a = t; end
        case 1
            cancel = (brake_pedal > 0.5) || (abs(tau) > 4 && clonic < 0.5 && grip < 1.5);
            if cancel
                st = 0;  vcnt = 0;  cool = t + 10;  buf(:) = 0;
            elseif t - t_a >= pv(13)
                st = 2;
            end
        case 2
            if t - t_a >= pv(6), st = 3; end
        case 3
            if v < 0.3, st = 4; end
    end
end

hung = (pv(8) == 4) && (t >= pv(9));          % host hang: goes silent
send = double(tick && pv(15) > 0.5 && ~hung);
dec = 0;
if st >= 3, dec = pv(7); end
hf = [send; st; dec; 1; 1];
F = double(st >= 1);
alert = double(st == 1);
dmode = md;
Pmax = Pm;
cls = cl * double(st >= 1);
ecall = double(st >= 2);                      % call placed when the alert goes unanswered
warn = wr;
state = st;
end

== matlab function CabinGuard_MATLAB_simulation/CabinGuard/Gw ==
  settings: updateMethod=DISCRETE  sampleTime=0.01
  data: t input; a_mrm output; hf input; att input; v input; pv input; gwp_out output; lk_on output; y_ref output; park_out output; alive_lost output; reject output; nrej_out output
function [a_mrm, gwp_out, lk_on, y_ref, park_out, alive_lost, reject, nrej_out] = fcn(t, hf, att, v, pv)
% ACTUATOR GATEWAY: the trusted boundary in front of the actuators.
%   Accepts a frame only if (authenticated AND fresh) AND phase order plausible AND
%   -4 <= decel <= 0. Host frames double as alive signal (300 ms timeout).
%   Host lost: nothing is actuated, unless a manoeuvre is already under way
%   (phase >= pv(11)), in which case the gateway completes the stop on its own.
Ts = 0.01;  JERK = 5;
persistent gwp a_out t_ok t_ph2 last_dec park nrej
if isempty(gwp)
    gwp = 0;  a_out = 0;  t_ok = 0;  t_ph2 = -1;  last_dec = 0;  park = false;  nrej = 0;
end
fr = zeros(5, 2);                             % column 1 host, column 2 attacker
fr(:, 1) = hf(1:5);
fr(:, 2) = att(1:5);
reject = 0;
for k = 1:2
    f = fr(:, k);
    if f(1) > 0.5
        ph = round(f(2));  dc = f(3);
        ok_auth = (f(4) > 0.5) && (f(5) > 0.5);
        ok_ph = (ph == gwp) || (ph == gwp + 1) || (ph == 0 && gwp == 1);
        ok_dc = (dc <= 0) && (dc >= -4);
        if ok_auth && ok_ph && ok_dc
            if ph ~= gwp
                gwp = ph;
                if ph == 2, t_ph2 = t; end
            end
            last_dec = dc;
            if k == 1, t_ok = t; end
        else
            reject = 1;  nrej = nrej + 1;
        end
    end
end
alive_lost = double((t - t_ok) > 0.3);

tgt = 0;
if alive_lost < 0.5
    if gwp >= 3, tgt = last_dec; end
else
    if gwp >= pv(11)
        if gwp >= 3
            tgt = min(last_dec, pv(7));
        elseif gwp == 2 && (t - t_ph2) >= (pv(6) - pv(13))
            gwp = 3;  tgt = pv(7);            % gateway-owned fallback timer
        end
    end
end
% taper the deceleration near standstill (no artificial stop jolt) and ramp it out once parked
if tgt < 0, tgt = tgt * min(1, 0.25 + max(v, 0)/2.0); end
if park, tgt = 0; end
da = max(-JERK*Ts, min(JERK*Ts, tgt - a_out));
a_out = a_out + da;
if gwp >= 3 && v < 0.1, park = true; end

a_mrm = a_out;                                % plant holds v = 0 while parked
gwp_out = gwp;
lk_on = double(pv(5) > 1.5 || (pv(5) > 0.5 && gwp >= 1));
y_ref = pv(12) * double(gwp >= 2);            % start the move to the shoulder at HAZARD
park_out = double(park);
nrej_out = nrej;
end
